simulink model "current_ctl_loop_task"  (R2023a)
settings: configuration reference "config" (kept outside this file)
libraries: mcbcontrolslib x4, simulink x4
settings Model: DataDictionary=model_config.sldd  Creator=huangcheng  LastModifiedBy=Administrator
settings ConfigSetRef: SourceName=config

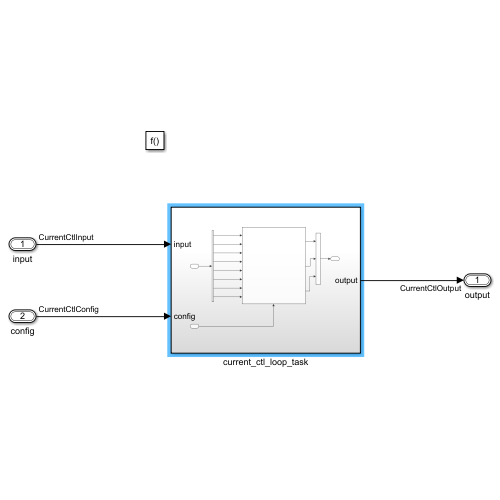
[thumbnail: Simulink's stored preview of the top-level diagram]
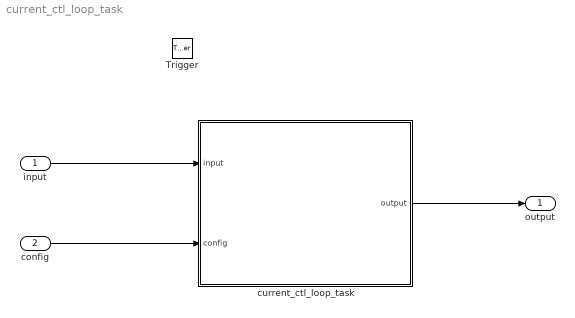
== system current_ctl_loop_task ==
  input : Inport  OutDataTypeStr=Bus: CurrentCtlInput  BusOutputAsStruct=on
  config : Inport  Port=2  OutDataTypeStr=Bus: CurrentCtlConfig  BusOutputAsStruct=on
  Trigger : TriggerPort  TriggerType=function-call  VariantControl=(inherit)  PortDimensions=1
  current_ctl_loop_task : Subsystem
  output : Outport  OutDataTypeStr=Bus: CurrentCtlOutput  BusOutputAsStruct=on
  wires:
  config/1 -> current_ctl_loop_task/2(config)
  input/1 -> current_ctl_loop_task/1(input)
  current_ctl_loop_task/1(output) -> output/1

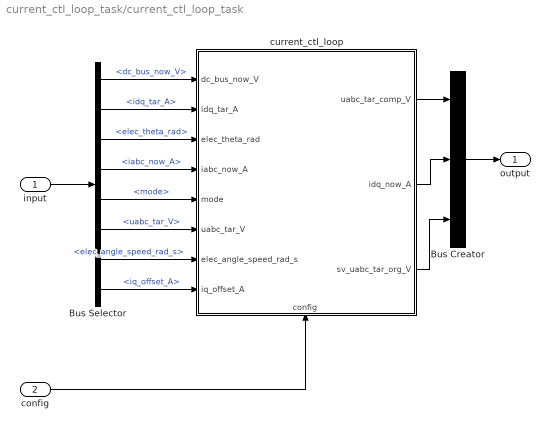
== system current_ctl_loop_task/current_ctl_loop_task ==
  input : Inport
  config : Inport  Port=2
  Bus Creator : BusCreator  Inputs=3  OutDataTypeStr=Bus: CurrentCtlOutput  NonVirtualBus=on
      settings: InheritFromInputs=off
  Bus Selector : BusSelector  OutputSignals=dc_bus_now_V,idq_tar_A,elec_theta_rad,iabc_now_A,mode,uabc_tar_V,elec_angle_speed_rad_s,iq_offset_A
  current_ctl_loop : Subsystem
      settings: PortSchema="{\"entries\":[{\"content\":{\"sides\":[{\"content\":{\"connectorIds\":[\"In1\",\"In2\",\"In3\",\"In4\",\"In5\",\"In6\",\"In7\",\"In8\"]},\"type\":\"ConnectorPlacement.EquallySpacedRectSide\",\"uuid\":\"b7a2fd29-5fd1-4133-99d1-58dff38eae7e\"},{\"content\":{\"connectorIds\":[\"Out1\",\"Out2\",\"Out3\"],\"side\":\"RIGHT\"},\"type\":\"ConnectorPlacement.EquallySpacedRectSide\",\"uuid\":\"301fc4cb-d0c0-4186-8441-a86c163f80af\"},{\"content\":{\"side\":\"TOP\"},\"type\":\"ConnectorPlacement.EquallySpacedRectSide\",\"uuid\":\"91a43a24-f62d-4f6e-b749-d43241765dd3\"},{\"content\":{\"connectorIds\":[\"In9\"],\"side\":\"BOTTOM\"},\"type\":\"ConnectorPlacement.EquallySpacedRectSide\",\"uuid\":\"8840c117-ad2e-4411-8f01-84a6a13e89bc\"}]},\"type\":\"ConnectorPlacement.EquallySpacedConnector\",\"uuid\":\"27fc35fe-1253-4901-beb3-8969cdc6c6b3\"}],\"packageUris\":[\"http://schema.mathworks.com/mf0/Connector/R2020b\"],\"version\":\"1.0\"}"
  output : Outport  OutDataTypeStr=Bus: CurrentCtlOutput
  wires:
  Bus Selector/6 -> current_ctl_loop/6(uabc_tar_V)  "<uabc_tar_V>"
  Bus Selector/3 -> current_ctl_loop/3(elec_theta_rad)  "<elec_theta_rad>"
  Bus Selector/2 -> current_ctl_loop/2(idq_tar_A)  "<idq_tar_A>"
  Bus Selector/1 -> current_ctl_loop/1(dc_bus_now_V)  "<dc_bus_now_V>"
  input/1 -> Bus Selector/1
  Bus Selector/4 -> current_ctl_loop/4(iabc_now_A)  "<iabc_now_A>"
  Bus Selector/5 -> current_ctl_loop/5(mode)  "<mode>"
  Bus Selector/7 -> current_ctl_loop/7(elec_angle_speed_rad_s)  "<elec_angle_speed_rad_s>"
  config/1 -> current_ctl_loop/9(config)
  current_ctl_loop/1(uabc_tar_comp_V) -> Bus Creator/1
  current_ctl_loop/2(idq_now_A) -> Bus Creator/2
  current_ctl_loop/3(sv_uabc_tar_org_V) -> Bus Creator/3
  Bus Creator/1 -> output/1
  Bus Selector/8 -> current_ctl_loop/8(iq_offset_A)  "<iq_offset_A>"

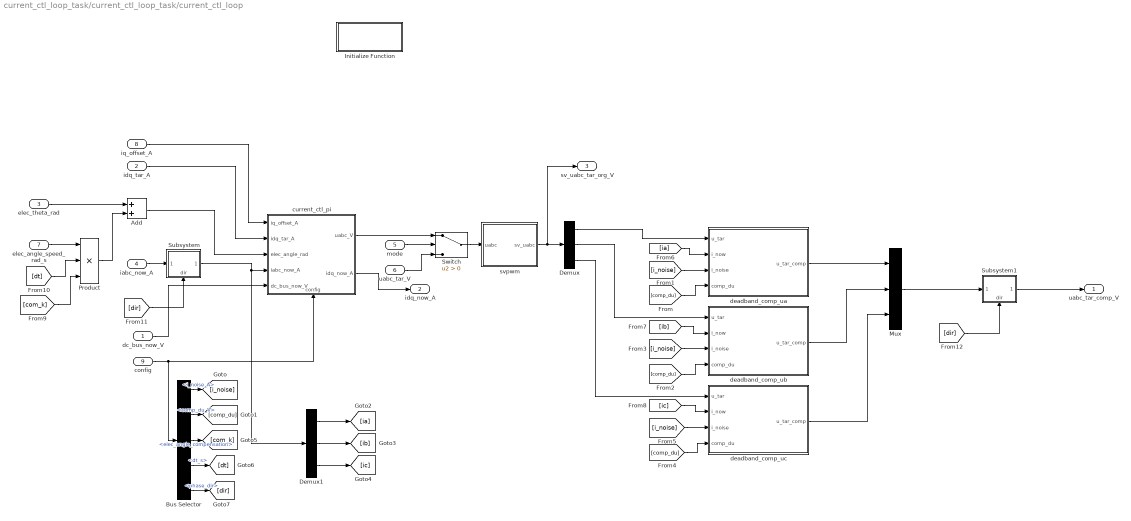
== system current_ctl_loop_task/current_ctl_loop_task/current_ctl_loop ==
  dc_bus_now_V : Inport
  idq_tar_A : Inport  Port=2
  elec_theta_rad : Inport  Port=3
  iabc_now_A : Inport  Port=4
  mode : Inport  Port=5
  uabc_tar_V : Inport  Port=6
  elec_angle_speed_rad_s : Inport  Port=7
  iq_offset_A : Inport  Port=8
  config : Inport  Port=9
  Add : Sum
  Bus Selector : BusSelector  OutputSignals=i_noise_A,comp_du_V,elec_angle_compensation,dt_s,phase_dir
  Demux : Demux  Outputs=3
  Demux1 : Demux  Outputs=3
  Initialize Function : Subsystem  TreatAsAtomicUnit=on
  Mux : Mux  Inputs=3
  Product : Product  Inputs=3
  Subsystem : Subsystem
      settings: PortSchema="{\"entries\":[{\"content\":{\"sides\":[{\"content\":{\"connectorIds\":[\"In1\"]},\"type\":\"ConnectorPlacement.EquallySpacedRectSide\",\"uuid\":\"99578d5e-51cd-4db8-8bee-4ee570f64834\"},{\"content\":{\"connectorIds\":[\"Out1\"],\"side\":\"RIGHT\"},\"type\":\"ConnectorPlacement.EquallySpacedRectSide\",\"uuid\":\"5ce2eafc-f891-4109-a15c-892f6316f510\"},{\"content\":{\"side\":\"TOP\"},\"type\":\"ConnectorPlacement.EquallySpacedRectSide\",\"uuid\":\"d11b8e50-530a-4fbe-aceb-a5cfb4b17408\"},{\"content\":{\"connectorIds\":[\"In2\"],\"side\":\"BOTTOM\"},\"type\":\"ConnectorPlacement.EquallySpacedRectSide\",\"uuid\":\"3560f0d8-2a2c-4c4e-b486-a040a021bd38\"}]},\"type\":\"ConnectorPlacement.EquallySpacedConnector\",\"uuid\":\"79e83196-5e7d-4b67-86e2-4808db3aa3ea\"}],\"packageUris\":[\"http://schema.mathworks.com/mf0/Connector/R2020b\"],\"version\":\"1.0\"}"
  Subsystem1 : Subsystem
      settings: PortSchema="{\"entries\":[{\"content\":{\"sides\":[{\"content\":{\"connectorIds\":[\"In1\"]},\"type\":\"ConnectorPlacement.EquallySpacedRectSide\",\"uuid\":\"99578d5e-51cd-4db8-8bee-4ee570f64834\"},{\"content\":{\"connectorIds\":[\"Out1\"],\"side\":\"RIGHT\"},\"type\":\"ConnectorPlacement.EquallySpacedRectSide\",\"uuid\":\"5ce2eafc-f891-4109-a15c-892f6316f510\"},{\"content\":{\"side\":\"TOP\"},\"type\":\"ConnectorPlacement.EquallySpacedRectSide\",\"uuid\":\"d11b8e50-530a-4fbe-aceb-a5cfb4b17408\"},{\"content\":{\"connectorIds\":[\"In2\"],\"side\":\"BOTTOM\"},\"type\":\"ConnectorPlacement.EquallySpacedRectSide\",\"uuid\":\"3560f0d8-2a2c-4c4e-b486-a040a021bd38\"}]},\"type\":\"ConnectorPlacement.EquallySpacedConnector\",\"uuid\":\"79e83196-5e7d-4b67-86e2-4808db3aa3ea\"}],\"packageUris\":[\"http://schema.mathworks.com/mf0/Connector/R2020b\"],\"version\":\"1.0\"}"
  Switch : Switch  Criteria=u2 > Threshold  SaturateOnIntegerOverflow=off  InputSameDT=off
  current_ctl_pi : Subsystem
      settings: PortSchema="{\"entries\":[{\"content\":{\"sides\":[{\"content\":{\"connectorIds\":[\"In1\",\"In2\",\"In3\",\"In4\",\"In5\"]},\"type\":\"ConnectorPlacement.EquallySpacedRectSide\",\"uuid\":\"130fac9a-5859-491f-9ebe-59afcce514ec\"},{\"content\":{\"connectorIds\":[\"Out1\",\"Out2\"],\"side\":\"RIGHT\"},\"type\":\"ConnectorPlacement.EquallySpacedRectSide\",\"uuid\":\"9816416b-9cc1-4c78-a5db-413ecd238268\"},{\"content\":{\"side\":\"TOP\"},\"type\":\"ConnectorPlacement.EquallySpacedRectSide\",\"uuid\":\"4217a915-d85c-4594-b57f-d0567f09ab46\"},{\"content\":{\"connectorIds\":[\"In6\"],\"side\":\"BOTTOM\"},\"type\":\"ConnectorPlacement.EquallySpacedRectSide\",\"uuid\":\"c99b6a34-fffa-47ce-9724-12be4ca5a9f3\"}]},\"type\":\"ConnectorPlacement.EquallySpacedConnector\",\"uuid\":\"02dddf2c-6dec-4098-832f-fa7f826aee20\"}],\"packageUris\":[\"http://schema.mathworks.com/mf0/Connector/R2020b\"],\"version\":\"1.0\"}"
  deadband_comp_ua : Subsystem  TreatAsAtomicUnit=on
  deadband_comp_ub : Subsystem  TreatAsAtomicUnit=on
  deadband_comp_uc : Subsystem  TreatAsAtomicUnit=on
  "svpwm " : MATLAB Function
  uabc_tar_comp_V : Outport
  idq_now_A : Outport  Port=2
  sv_uabc_tar_org_V : Outport  Port=3
  wires:
  Demux/3 -> deadband_comp_uc/1(u_tar)
  deadband_comp_ub/1(u_tar_comp) -> Mux/2
  Demux/2 -> deadband_comp_ub/1(u_tar)
  dc_bus_now_V/1 -> current_ctl_pi/5(dc_bus_now_V)
  Subsystem/1(iabc_real_now_A) -> Demux1/1, current_ctl_pi/4(iabc_now_A)
  current_ctl_pi/2(idq_now_A) -> idq_now_A/1
  deadband_comp_ua/1(u_tar_comp) -> Mux/1
  deadband_comp_uc/1(u_tar_comp) -> Mux/3
  Demux/1 -> deadband_comp_ua/1(u_tar)
  idq_tar_A/1 -> current_ctl_pi/2(idq_tar_A)
  config/1 -> Bus Selector/1, current_ctl_pi/6(config)
  Bus Selector/1 -> [i_noise]  "<i_noise_A>"
  Bus Selector/2 -> [comp_du]  "<comp_du_V>"
  [i_noise] -> deadband_comp_ua/3(i_noise)
  [comp_du] -> deadband_comp_ua/4(comp_du)
  [i_noise] -> deadband_comp_ub/3(i_noise)
  [comp_du] -> deadband_comp_ub/4(comp_du)
  [i_noise] -> deadband_comp_uc/3(i_noise)
  [comp_du] -> deadband_comp_uc/4(comp_du)
  mode/1 -> Switch/2
  uabc_tar_V/1 -> Switch/3
  Switch/1 -> "svpwm "/1(uabc)
  Demux1/1 -> [ia]
  Demux1/2 -> [ib]
  Demux1/3 -> [ic]
  [ia] -> deadband_comp_ua/2(i_now)
  [ib] -> deadband_comp_ub/2(i_now)
  [ic] -> deadband_comp_uc/2(i_now)
  Bus Selector/3 -> [com_k]  "<elec_angle_compensation>"
  Bus Selector/4 -> [dt]  "<dt_s>"
  elec_angle_speed_rad_s/1 -> Product/1
  [dt] -> Product/2
  [com_k] -> Product/3
  elec_theta_rad/1 -> Add/1
  Add/1 -> current_ctl_pi/3(elec_angle_rad)
  Product/1 -> Add/2
  Bus Selector/5 -> [dir]  "<phase_dir>"
  iabc_now_A/1 -> Subsystem/1(iabc_now_A)
  [dir] -> Subsystem/2(dir)
  [dir] -> Subsystem1/2(dir)
  Mux/1 -> Subsystem1/1(uabc_now_V)
  Subsystem1/1(uabc_real_now_V) -> uabc_tar_comp_V/1
  current_ctl_pi/1(uabc_V) -> Switch/1
  "svpwm "/1(sv_uabc) -> sv_uabc_tar_org_V/1, Demux/1
  iq_offset_A/1 -> current_ctl_pi/1(iq_offset_A)

== system current_ctl_loop_task/current_ctl_loop_task/current_ctl_loop/Initialize Function ==
  Constant1 : Constant  Value=0  OutDataTypeStr=single
  Constant2 : Constant  Value=0  OutDataTypeStr=single
  Event Listener : EventListener  DisableCoverage=on  EventName=reset
  State Writer : StateWriter  StateOwnerBlock=../../current_ctl_pi/current_ctl_pi/id_pi_ctl/Delay  StateName=id_ki_int
  State Writer1 : StateWriter  StateOwnerBlock=../../current_ctl_pi/current_ctl_pi/iq_pi_ctl/Delay  StateName=iq_ki_int
  wires:
  Constant1/1 -> State Writer/1
  Constant2/1 -> State Writer1/1

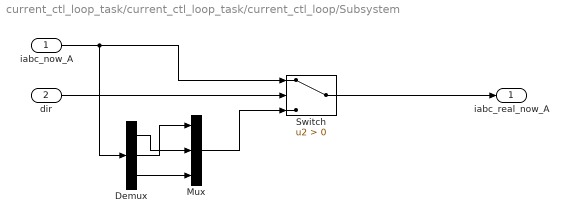
== system current_ctl_loop_task/current_ctl_loop_task/current_ctl_loop/Subsystem ==
  iabc_now_A : Inport
  dir : Inport  Port=2
  Demux : Demux  Outputs=3
  Mux : Mux  Inputs=3
  Switch : Switch  Criteria=u2 > Threshold  SaturateOnIntegerOverflow=off  InputSameDT=off
  iabc_real_now_A : Outport
  wires:
  dir/1 -> Switch/2
  iabc_now_A/1 -> Demux/1, Switch/1
  Switch/1 -> iabc_real_now_A/1
  Demux/3 -> Mux/3
  Demux/1 -> Mux/2
  Demux/2 -> Mux/1
  Mux/1 -> Switch/3

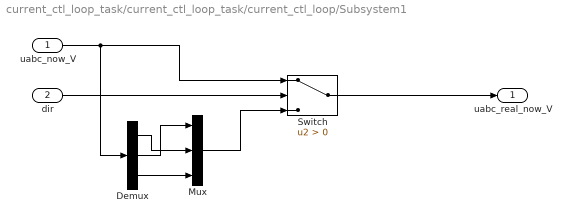
== system current_ctl_loop_task/current_ctl_loop_task/current_ctl_loop/Subsystem1 ==
  uabc_now_V : Inport
  dir : Inport  Port=2
  Demux : Demux  Outputs=3
  Mux : Mux  Inputs=3
  Switch : Switch  Criteria=u2 > Threshold  SaturateOnIntegerOverflow=off  InputSameDT=off
  uabc_real_now_V : Outport
  wires:
  dir/1 -> Switch/2
  uabc_now_V/1 -> Demux/1, Switch/1
  Switch/1 -> uabc_real_now_V/1
  Demux/3 -> Mux/3
  Demux/1 -> Mux/2
  Demux/2 -> Mux/1
  Mux/1 -> Switch/3

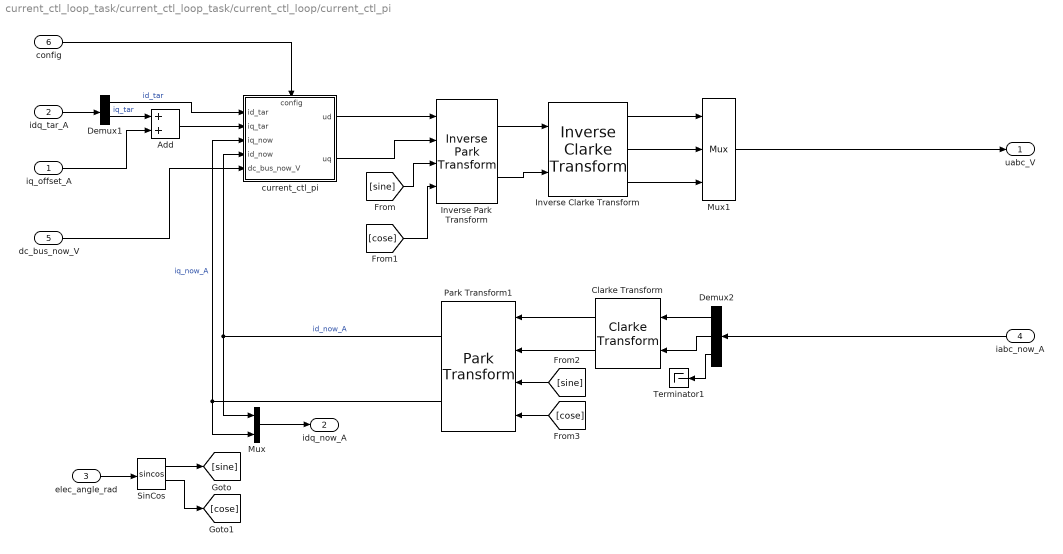
== system current_ctl_loop_task/current_ctl_loop_task/current_ctl_loop/current_ctl_pi ==
  iq_offset_A : Inport
  idq_tar_A : Inport  Port=2  OutDataTypeStr=single  PortDimensions=2
  elec_angle_rad : Inport  Port=3
  iabc_now_A : Inport  Port=4  PortDimensions=3
  dc_bus_now_V : Inport  Port=5
  config : Inport  Port=6
  Add : Sum
  Clarke Transform : mcbcontrolslib/Clarke Transform  VariantControl=Variant2
  Demux1 : Demux  Outputs=2
  Demux2 : Demux  Outputs=3
  Inverse Clarke Transform : mcbcontrolslib/Inverse Clarke Transform
      settings: LibrarySourceBlock=mcbhdllib/Controls/Math Transforms/Inverse Clarke Transform
  Inverse Park Transform : mcbcontrolslib/Inverse Park Transform  AxisAlignment=D-axis
  Mux : Mux  Inputs=2
  Mux1 : Mux  Inputs=3
  Park Transform1 : mcbcontrolslib/Park Transform  AxisAlignment=D-axis
  SinCos : Trigonometry  Operator=sincos  OutputSignalType=real
  Terminator1 : Terminator
  current_ctl_pi : Subsystem  SystemSampleTime=5e-5
      settings: PortSchema="{\"entries\":[{\"content\":{\"sides\":[{\"content\":{\"connectorIds\":[\"In1\",\"In2\",\"In3\",\"In4\",\"In5\"]},\"type\":\"ConnectorPlacement.EquallySpacedRectSide\",\"uuid\":\"867e764e-d5fb-403b-b180-f9d74fa69a85\"},{\"content\":{\"connectorIds\":[\"Out1\",\"Out2\"],\"side\":\"RIGHT\"},\"type\":\"ConnectorPlacement.EquallySpacedRectSide\",\"uuid\":\"c4ac5134-4a96-4227-ad7c-5f214280f25c\"},{\"content\":{\"connectorIds\":[\"In6\"],\"side\":\"TOP\"},\"type\":\"ConnectorPlacement.EquallySpacedRectSide\",\"uuid\":\"8f8549d1-471d-4d0b-8fc2-e080d793ab5b\"}]},\"type\":\"ConnectorPlacement.EquallySpacedConnector\",\"uuid\":\"68a57a21-5f6c-48c6-8161-083643c15cbb\"}],\"packageUris\":[\"http://schema.mathworks.com/mf0/Connector/R2020b\"],\"version\":\"1.0\"}"
  uabc_V : Outport  OutDataTypeStr=single  PortDimensions=3
  idq_now_A : Outport  Port=2
  wires:
  Park Transform1/2 -> current_ctl_pi/3(iq_now), Mux/2  "iq_now_A"
  idq_tar_A/1 -> Demux1/1
  Park Transform1/1 -> current_ctl_pi/4(id_now), Mux/1  "id_now_A"
  Demux1/1 -> current_ctl_pi/1(id_tar)  "id_tar"
  iabc_now_A/1 -> Demux2/1
  Mux/1 -> idq_now_A/1
  dc_bus_now_V/1 -> current_ctl_pi/5(dc_bus_now_V)
  config/1 -> current_ctl_pi/6(config)
  elec_angle_rad/1 -> SinCos/1
  SinCos/1 -> [sine]
  SinCos/2 -> [cose]
  Inverse Park Transform/1 -> Inverse Clarke Transform/1
  Inverse Park Transform/2 -> Inverse Clarke Transform/2
  current_ctl_pi/1(ud) -> Inverse Park Transform/1
  current_ctl_pi/2(uq) -> Inverse Park Transform/2
  [sine] -> Inverse Park Transform/3
  [cose] -> Inverse Park Transform/4
  Demux2/3 -> Terminator1/1
  Demux2/1 -> Clarke Transform/1
  Demux2/2 -> Clarke Transform/2
  Clarke Transform/1 -> Park Transform1/1
  Clarke Transform/2 -> Park Transform1/2
  [sine] -> Park Transform1/3
  [cose] -> Park Transform1/4
  Inverse Clarke Transform/2 -> Mux1/2
  Inverse Clarke Transform/1 -> Mux1/1
  Inverse Clarke Transform/3 -> Mux1/3
  Mux1/1 -> uabc_V/1
  iq_offset_A/1 -> Add/2
  Demux1/2 -> Add/1  "iq_tar"
  Add/1 -> current_ctl_pi/2(iq_tar)

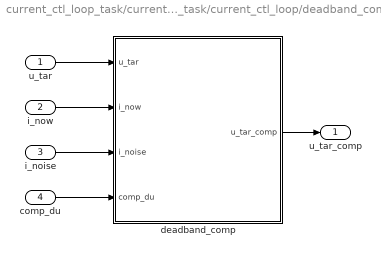
== system current_ctl_loop_task/current_ctl_loop_task/current_ctl_loop/deadband_comp_ua ==
  u_tar : Inport
  i_now : Inport  Port=2
  i_noise : Inport  Port=3
  comp_du : Inport  Port=4
  deadband_comp : MATLAB Function  TreatAsAtomicUnit=on
  u_tar_comp : Outport
  wires:
  u_tar/1 -> deadband_comp/1(u_tar)
  deadband_comp/1(u_tar_comp) -> u_tar_comp/1
  i_noise/1 -> deadband_comp/3(i_noise)
  i_now/1 -> deadband_comp/2(i_now)
  comp_du/1 -> deadband_comp/4(comp_du)

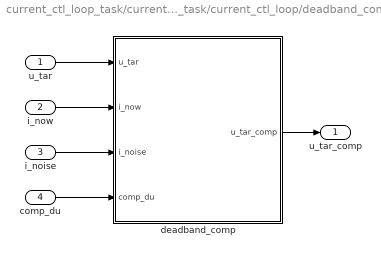
== system current_ctl_loop_task/current_ctl_loop_task/current_ctl_loop/deadband_comp_ub ==
  u_tar : Inport
  i_now : Inport  Port=2
  i_noise : Inport  Port=3
  comp_du : Inport  Port=4
  deadband_comp : MATLAB Function  TreatAsAtomicUnit=on
  u_tar_comp : Outport
  wires:
  u_tar/1 -> deadband_comp/1(u_tar)
  deadband_comp/1(u_tar_comp) -> u_tar_comp/1
  i_noise/1 -> deadband_comp/3(i_noise)
  i_now/1 -> deadband_comp/2(i_now)
  comp_du/1 -> deadband_comp/4(comp_du)

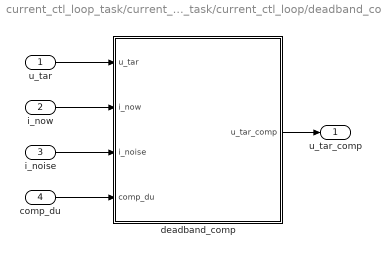
== system current_ctl_loop_task/current_ctl_loop_task/current_ctl_loop/deadband_comp_uc ==
  u_tar : Inport
  i_now : Inport  Port=2
  i_noise : Inport  Port=3
  comp_du : Inport  Port=4
  deadband_comp : MATLAB Function  TreatAsAtomicUnit=on
  u_tar_comp : Outport
  wires:
  comp_du/1 -> deadband_comp/4(comp_du)
  i_now/1 -> deadband_comp/2(i_now)
  i_noise/1 -> deadband_comp/3(i_noise)
  deadband_comp/1(u_tar_comp) -> u_tar_comp/1
  u_tar/1 -> deadband_comp/1(u_tar)

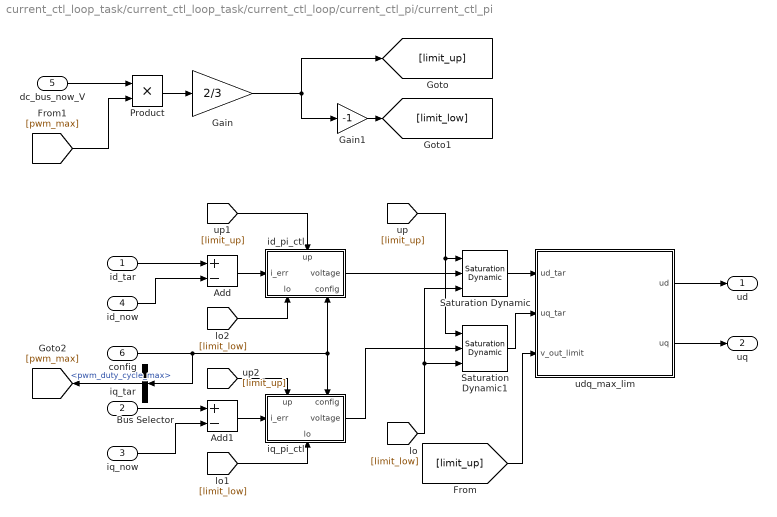
== system current_ctl_loop_task/current_ctl_loop_task/current_ctl_loop/current_ctl_pi/current_ctl_pi ==
  id_tar : Inport
  iq_tar : Inport  Port=2
  iq_now : Inport  Port=3
  id_now : Inport  Port=4
  dc_bus_now_V : Inport  Port=5
  config : Inport  Port=6
  Add : Sum  Inputs=+-
  Add1 : Sum  Inputs=+-
  Bus Selector : BusSelector  OutputSignals=pwm_duty_cycle_max
  Gain : Gain  Gain=2/3
  Gain1 : Gain  Gain=-1
  Product : Product
  Saturation Dynamic : simulink/Discontinuities/Saturation Dynamic  OutMin=[]  OutMax=[]  OutDataTypeStr=Inherit: Same as second input  OutDataType=fixdt(1, 16)  OutScaling=2^-10  DoSatur=off
  Saturation Dynamic1 : simulink/Discontinuities/Saturation Dynamic  OutMin=[]  OutMax=[]  OutDataTypeStr=Inherit: Same as second input  OutDataType=fixdt(1, 16)  OutScaling=2^-10  DoSatur=off
  id_pi_ctl : Subsystem
      settings: PortSchema="{\"entries\":[{\"content\":{\"sides\":[{\"content\":{\"connectorIds\":[\"In1\"]},\"type\":\"ConnectorPlacement.EquallySpacedRectSide\",\"uuid\":\"c1844c88-1674-45a0-9162-ed878ab5f875\"},{\"content\":{\"connectorIds\":[\"Out1\"],\"side\":\"RIGHT\"},\"type\":\"ConnectorPlacement.EquallySpacedRectSide\",\"uuid\":\"e31a8f95-4a38-441d-8910-e435a2d47625\"},{\"content\":{\"connectorIds\":[\"In2\"],\"side\":\"TOP\"},\"type\":\"ConnectorPlacement.EquallySpacedRectSide\",\"uuid\":\"19790e4f-e49d-4c5f-9b24-5e7784090165\"},{\"content\":{\"connectorIds\":[\"In3\",\"In4\"],\"side\":\"BOTTOM\"},\"type\":\"ConnectorPlacement.EquallySpacedRectSide\",\"uuid\":\"52b1564c-0973-4838-ba98-4979f0071d24\"}]},\"type\":\"ConnectorPlacement.EquallySpacedConnector\",\"uuid\":\"b4def285-36eb-4924-b022-daf3bf206908\"}],\"packageUris\":[\"http://schema.mathworks.com/mf0/Connector/R2020b\"],\"version\":\"1.0\"}"
  iq_pi_ctl : Subsystem
      settings: PortSchema="{\"entries\":[{\"content\":{\"sides\":[{\"content\":{\"connectorIds\":[\"In1\"]},\"type\":\"ConnectorPlacement.EquallySpacedRectSide\",\"uuid\":\"c1844c88-1674-45a0-9162-ed878ab5f875\"},{\"content\":{\"connectorIds\":[\"Out1\"],\"side\":\"RIGHT\"},\"type\":\"ConnectorPlacement.EquallySpacedRectSide\",\"uuid\":\"e31a8f95-4a38-441d-8910-e435a2d47625\"},{\"content\":{\"connectorIds\":[\"In2\",\"In3\"],\"side\":\"TOP\"},\"type\":\"ConnectorPlacement.EquallySpacedRectSide\",\"uuid\":\"19790e4f-e49d-4c5f-9b24-5e7784090165\"},{\"content\":{\"connectorIds\":[\"In4\"],\"side\":\"BOTTOM\"},\"type\":\"ConnectorPlacement.EquallySpacedRectSide\",\"uuid\":\"52b1564c-0973-4838-ba98-4979f0071d24\"}]},\"type\":\"ConnectorPlacement.EquallySpacedConnector\",\"uuid\":\"b4def285-36eb-4924-b022-daf3bf206908\"}],\"packageUris\":[\"http://schema.mathworks.com/mf0/Connector/R2020b\"],\"version\":\"1.0\"}"
  udq_max_lim : MATLAB Function  TreatAsAtomicUnit=on
  ud : Outport
  uq : Outport  Port=2
  wires:
  Add/1 -> id_pi_ctl/1(i_err)
  id_tar/1 -> Add/1
  id_now/1 -> Add/2
  iq_tar/1 -> Add1/1
  Add1/1 -> iq_pi_ctl/1(i_err)
  iq_now/1 -> Add1/2
  id_pi_ctl/1(voltage) -> Saturation Dynamic/2
  iq_pi_ctl/1(voltage) -> Saturation Dynamic1/2
  Saturation Dynamic/1 -> udq_max_lim/1(ud_tar)
  Saturation Dynamic1/1 -> udq_max_lim/2(uq_tar)
  [limit_up] -> udq_max_lim/3(v_out_limit)
  Gain/1 -> Gain1/1, [limit_up]
  Gain1/1 -> [limit_low]
  [limit_up] -> Saturation Dynamic1/1, Saturation Dynamic/1
  [limit_low] -> Saturation Dynamic1/3, Saturation Dynamic/3
  [limit_low] -> iq_pi_ctl/4(lo)
  [limit_up] -> id_pi_ctl/2(up)
  [limit_up] -> iq_pi_ctl/2(up)
  [limit_low] -> id_pi_ctl/3(lo)
  config/1 -> Bus Selector/1, id_pi_ctl/4(config), iq_pi_ctl/3(config)
  Bus Selector/1 -> [pwm_max]  "<pwm_duty_cycle_max>"
  Product/1 -> Gain/1
  dc_bus_now_V/1 -> Product/1
  [pwm_max] -> Product/2
  udq_max_lim/1(ud) -> ud/1
  udq_max_lim/2(uq) -> uq/1

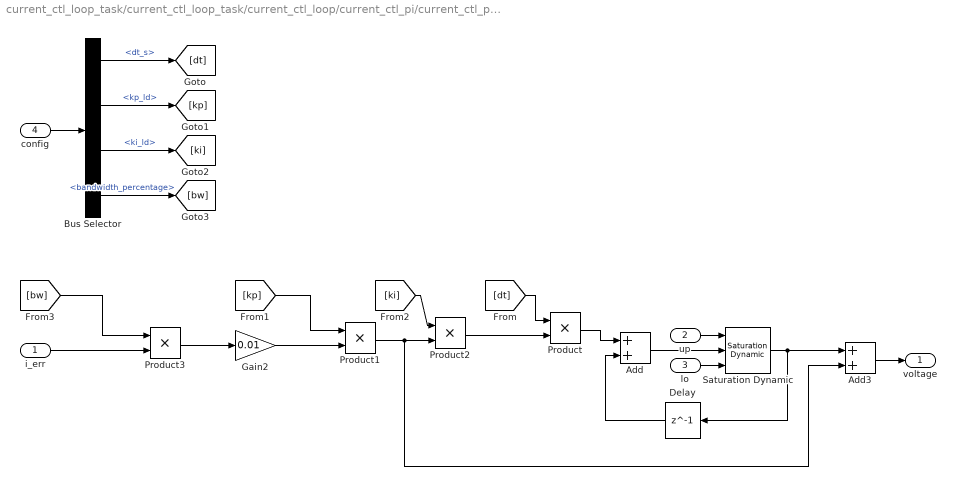
== system current_ctl_loop_task/current_ctl_loop_task/current_ctl_loop/current_ctl_pi/current_ctl_pi/id_pi_ctl ==
  i_err : Inport
  up : Inport  Port=2
  lo : Inport  Port=3
  config : Inport  Port=4
  Add : Sum
  Add3 : Sum
  Bus Selector : BusSelector  OutputSignals=dt_s,kp_ld,ki_ld,bandwidth_percentage
  Delay : Delay  DelayLength=1  StateName=id_ki_int
  Gain2 : Gain  Gain=0.01
  Product{,1..3} (4 alike) : Product
  Saturation Dynamic : simulink/Discontinuities/Saturation Dynamic  OutMin=[]  OutMax=[]  OutDataTypeStr=Inherit: Same as second input  OutDataType=fixdt(1, 16)  OutScaling=2^-10  DoSatur=off
  voltage : Outport
  wires:
  Product2/1 -> Product/2
  Add3/1 -> voltage/1
  Product1/1 -> Product2/2, Add3/2
  i_err/1 -> Product3/2
  Saturation Dynamic/1 -> Delay/1, Add3/1
  Product/1 -> Add/1
  Delay/1 -> Add/2
  Add/1 -> Saturation Dynamic/2
  up/1 -> Saturation Dynamic/1
  lo/1 -> Saturation Dynamic/3
  config/1 -> Bus Selector/1
  Bus Selector/1 -> [dt]  "<dt_s>"
  [dt] -> Product/1
  Bus Selector/2 -> [kp]  "<kp_ld>"
  Bus Selector/3 -> [ki]  "<ki_ld>"
  Bus Selector/4 -> [bw]  "<bandwidth_percentage>"
  [kp] -> Product1/1
  [ki] -> Product2/1
  Product3/1 -> Gain2/1
  Gain2/1 -> Product1/2
  [bw] -> Product3/1

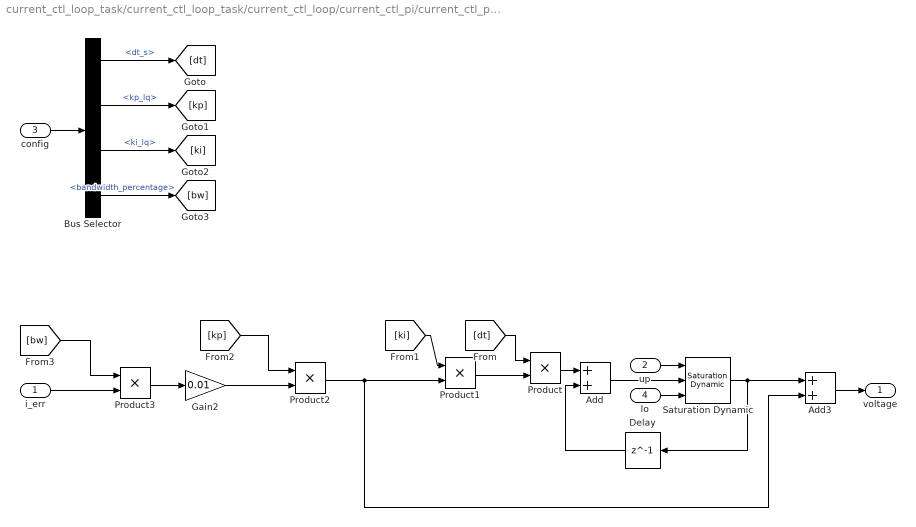
== system current_ctl_loop_task/current_ctl_loop_task/current_ctl_loop/current_ctl_pi/current_ctl_pi/iq_pi_ctl ==
  i_err : Inport
  up : Inport  Port=2
  config : Inport  Port=3
  lo : Inport  Port=4
  Add : Sum
  Add3 : Sum
  Bus Selector : BusSelector  OutputSignals=dt_s,kp_lq,ki_lq,bandwidth_percentage
  Delay : Delay  DelayLength=1  StateName=iq_ki_int
  Gain2 : Gain  Gain=0.01
  Product{,1..3} (4 alike) : Product
  Saturation Dynamic : simulink/Discontinuities/Saturation Dynamic  OutMin=[]  OutMax=[]  OutDataTypeStr=Inherit: Same as second input  OutDataType=fixdt(1, 16)  OutScaling=2^-10  DoSatur=off
  voltage : Outport
  wires:
  lo/1 -> Saturation Dynamic/3
  up/1 -> Saturation Dynamic/1
  Add/1 -> Saturation Dynamic/2
  Delay/1 -> Add/2
  Product/1 -> Add/1
  Saturation Dynamic/1 -> Add3/1, Delay/1
  i_err/1 -> Product3/2
  Product2/1 -> Product1/2, Add3/2
  Add3/1 -> voltage/1
  Product1/1 -> Product/2
  config/1 -> Bus Selector/1
  Bus Selector/3 -> [ki]  "<ki_lq>"
  Bus Selector/2 -> [kp]  "<kp_lq>"
  Bus Selector/4 -> [bw]  "<bandwidth_percentage>"
  Bus Selector/1 -> [dt]  "<dt_s>"
  [dt] -> Product/1
  [ki] -> Product1/1
  [kp] -> Product2/1
  Product3/1 -> Gain2/1
  [bw] -> Product3/1
  Gain2/1 -> Product2/2

== matlab function current_ctl_loop_task/current_ctl_loop/deadband_comp_ub/deadband_comp ==
  data: u_tar input; u_tar_comp output; i_now input; i_noise input; comp_du input
function u_tar_comp = deadband_comp(u_tar, i_now, i_noise, comp_du)
if i_noise < 0.00001
    u_tar_comp = single(0);
    return;  %入参  i_noise 必须 > 0.00001  是正数
end

du = single(0);  %补偿电压大小
line_range = i_noise * single(2);  %线性区域范围
k = comp_du / line_range;  %线性补偿斜率


if i_now <= line_range && i_now >= -line_range  % 在线性补偿范围内
    du = k * i_now;
else  %在非线性范围
    if i_now > single(0)
        du = comp_du;
    else
        du = -comp_du;    
    end
end

u_tar_comp = u_tar + du;

== matlab function current_ctl_loop_task/current_ctl_loop/deadband_comp_ua/deadband_comp ==
  data: u_tar input; u_tar_comp output; i_now input; i_noise input; comp_du input
function u_tar_comp = deadband_comp(u_tar, i_now, i_noise, comp_du)
if i_noise < 0.00001
    u_tar_comp = single(0);
    return;  %入参  i_noise 必须 > 0.00001  是正数
end

du = single(0);  %补偿电压大小
line_range = i_noise * single(2);  %线性区域范围
k = comp_du / line_range;  %线性补偿斜率


if i_now <= line_range && i_now >= -line_range  % 在线性补偿范围内
    du = k * i_now;
else  %在非线性范围
    if i_now > single(0)
        du = comp_du;
    else
        du = -comp_du;    
    end
end

u_tar_comp = u_tar + du;

== matlab function current_ctl_loop_task/current_ctl_loop/deadband_comp_uc/deadband_comp ==
  data: u_tar input; u_tar_comp output; i_now input; i_noise input; comp_du input
function u_tar_comp = deadband_comp(u_tar, i_now, i_noise, comp_du)
if i_noise < 0.00001
    u_tar_comp = single(0);
    return;  %入参  i_noise 必须 > 0.00001  是正数
end

du = single(0);  %补偿电压大小
line_range = i_noise * single(2);  %线性区域范围
k = comp_du / line_range;  %线性补偿斜率


if i_now <= line_range && i_now >= -line_range  % 在线性补偿范围内
    du = k * i_now;
else  %在非线性范围
    if i_now > single(0)
        du = comp_du;
    else
        du = -comp_du;    
    end
end

u_tar_comp = u_tar + du;

== matlab function current_ctl_loop_task/current_ctl_loop/current_ctl_pi/current_ctl_pi/udq_max_lim ==
  data: ud_tar input; ud output; uq_tar input; v_out_limit input; uq output
function [ud, uq] = udq_max_lim(ud_tar, uq_tar, v_out_limit)

uq_temp = single(v_out_limit^2-ud_tar^2);

if(uq_temp >= 0)
    uq_max = single(sqrt(uq_temp));
else
    uq_max = single(0);
end

if(uq_tar > uq_max)
    uq_tar = uq_max;
elseif(uq_tar < -uq_max)
    uq_tar = -uq_max;    
end

ud = single(ud_tar);
uq = single(uq_tar);

== matlab function current_ctl_loop_task/current_ctl_loop/svpwm  ==
  data: uabc input; sv_uabc output
function sv_uabc  = svpwm_genrate(uabc)
%最大值最小值法
va = single(uabc(1));
vb = single(uabc(2));
vc = single(uabc(3));
sv_uabc = single(zeros(3,1));

if va>vb
    vmax = va;
    vmin = vb;
else
    vmax = vb;
    vmin = va;
end

if vc>vmax
    vmax = vc;
elseif vc<vmin
    vmin = vc;
end

vcom = 0.5*(vmax+vmin);

ua = va-vcom;
ub = vb-vcom;
uc = vc-vcom;

sv_uabc(1) = single(ua);
sv_uabc(2) = single(ub);
sv_uabc(3) = single(uc);
